simulink subsystem "ConfiguredSimulinkPlantModel"  (R2025b)
settings: Solver=VariableStepAuto  StartTime=0.0  StopTime=10.0  RelTol=1e-3
undefined symbols (not defined in the file or in its folder): PlntTrnsfrCaseAxlSpdLock, PlntTrnsfrCaseTrqSplitRatio
libraries: simulink x2
settings Model: ModifiedByFormat=The MathWorks, Inc.  Creator=The MathWorks, Inc.  LastModifiedBy=The MathWorks, Inc.
settings RTWCC: GPUComputeCapability=3.5

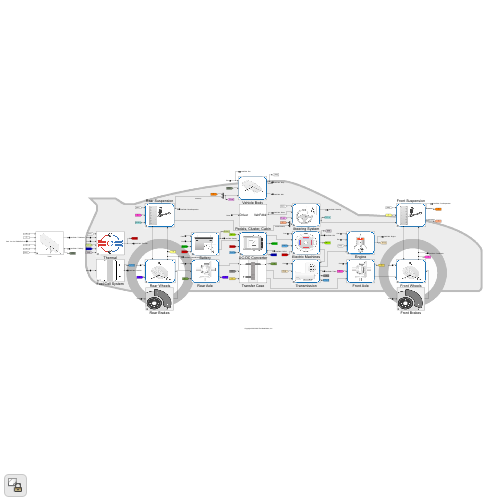
[thumbnail: Simulink's stored preview of the top-level diagram]
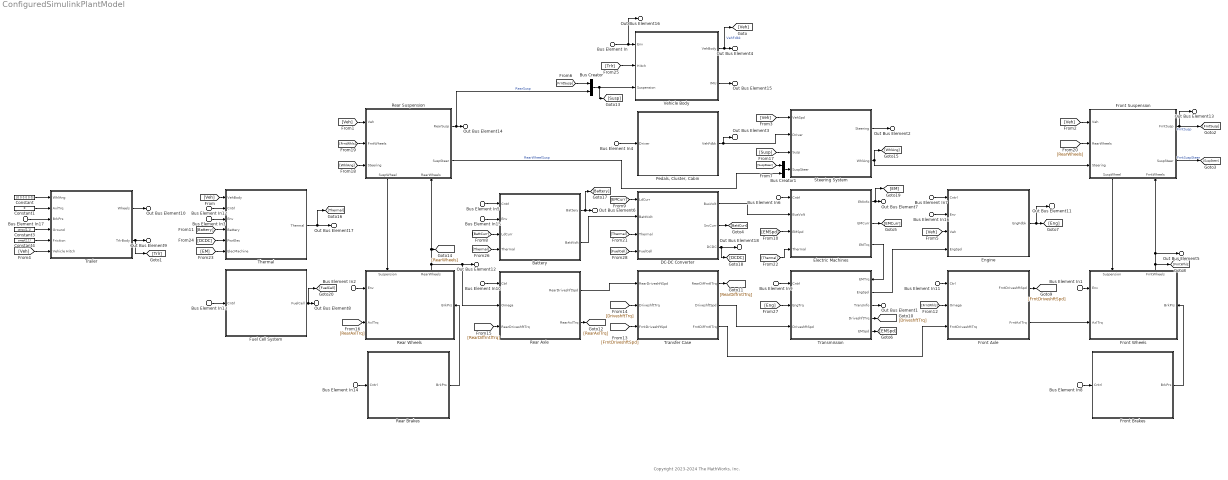
== system ConfiguredSimulinkPlantModel ==
  note: Copyright 2023-2024 The MathWorks, Inc.
  Bus Element In{,1..3,15..16} (6 alike) : Inport  PortName=Env
  Bus Element In4 : Inport  Port=2  PortName=Driver
  Bus Element In{5..14} (10 alike) : Inport  Port=3  PortName=Cntrl
  Bus Element In17 : Inport  Port=3  PortName=Cntrl  Element=Vcu.VcuTrlrBrkPrsCmd
  Battery : Subsystem  Variant=on  VariantChoicesSpecifier={'BatteryMapped'}  VariantControlMode=label  VariantControl=Battery  LabelModeActiveChoice=BatteryMapped
      mask Display: image('Battery.png'); % Use "Edit Image" on toolstrip to change.
  Bus Creator : BusCreator  Inputs=2
  Bus Creator1 : BusCreator  Inputs=2
  Constant : Constant  Value=[0 0 0 0 0 0]
  Constant1 : Constant  Value=0
  Constant3 : Constant  Value=zeros(2,1)
  Constant4 : Constant  Value=ones(2,1)
  DC-DC Converter : Subsystem  Variant=on  VariantChoicesSpecifier={'HVDCPassThrough'}  VariantControlMode=label  VariantControl=DC-DC Converter  LabelModeActiveChoice=HVDCPassThrough
      mask Display: image('DCDCConverter.png'); % Use "Edit Image" on toolstrip to change.
  Electric Machines : Subsystem  Variant=on  VariantChoicesSpecifier={'s2EM'}  VariantControlMode=label  VariantControl=Electric Machines  LabelModeActiveChoice=s2EM
      mask Display: image('Motor.png'); % Use "Edit Image" on toolstrip to change.
  Engine : Subsystem  Variant=on  VariantChoicesSpecifier={'SiMappedEngine'}  VariantControlMode=label  VariantControl=Engine  LabelModeActiveChoice=SiMappedEngine
      mask Display: image('Engine.png');
  Front Axle : Subsystem
      mask Display: image('OpenDifferential.png');
  Front Brakes : Subsystem  Variant=on  VariantControlMode=label  LabelModeActiveChoice=BrakingHydraulics
      mask Display: image('Caliper.png');
  Front Suspension : Subsystem  Variant=on  VariantChoicesSpecifier={'NoSuspensionFront'}  VariantControlMode=label  VariantControl=Front Suspension  LabelModeActiveChoice=NoSuspensionFront
      settings: PortSchema="{\"entries\":[{\"content\":{\"sides\":[{\"content\":{\"connectorIds\":[\"In1\",\"In2\",\"In3\"]},\"type\":\"ConnectorPlacement.EquallySpacedRectSide\",\"uuid\":\"03d471f7-20fa-4f88-95ae-1ed5ac0b2add\"},{\"content\":{\"connectorIds\":[\"Out1\",\"Out2\"],\"side\":\"RIGHT\"},\"type\":\"ConnectorPlacement.EquallySpacedRectSide\",\"uuid\":\"9ad6c778-1a7a-40eb-a466-797c67a1b13b\"},{\"content\":{\"side\":\"TOP\"},\"type\":\"ConnectorPlacement.EquallySpacedRectSide\",\"uuid\":\"82e0e713-e0a4-4b6c-9efd-1ca5e9a7cc75\"},{\"content\":{\"connectorIds\":[\"Out3\",\"In4\"],\"side\":\"BOTTOM\"},\"type\":\"ConnectorPlacement.EquallySpacedRectSide\",\"uuid\":\"217f9025-16e9-443b-9e91-f4a978a2b175\"}]},\"type\":\"ConnectorPlacement.EquallySpacedConnector\",\"uuid\":\"962b9c26-d5a5-4e4a-bd3b-22a258cb5c30\"}],\"packageUris\":[\"http://schema.mathworks.com/mf0/Connector/R2020b\"],\"version\":\"1.0\"}"
      mask Display: image('SimpleSusp.png'); % Use "Edit Image" on toolstrip to change.
  Front Wheels : Subsystem  Variant=on  VariantChoicesSpecifier={'MFTiresLongitudinalFront'}  VariantControlMode=label  VariantControl=Front Wheels  LabelModeActiveChoice=MFTiresLongitudinalFront
      settings: PortSchema="{\"entries\":[{\"content\":{\"sides\":[{\"content\":{\"connectorIds\":[\"In1\",\"In2\"]},\"type\":\"ConnectorPlacement.EquallySpacedRectSide\",\"uuid\":\"acc304d9-256c-4d8c-a59c-fdc4678acde8\"},{\"content\":{\"connectorIds\":[\"In4\"],\"side\":\"RIGHT\"},\"type\":\"ConnectorPlacement.EquallySpacedRectSide\",\"uuid\":\"17734490-d6e0-42a1-ab4b-fb468dc96262\"},{\"content\":{\"connectorIds\":[\"In3\",\"Out1\"],\"side\":\"TOP\"},\"type\":\"ConnectorPlacement.EquallySpacedRectSide\",\"uuid\":\"b3a5b678-2424-47a9-9e4a-20883a25a01f\"}]},\"type\":\"ConnectorPlacement.EquallySpacedConnector\",\"uuid\":\"2051c4aa-303b-4f53-baee-0d5c16c2d89d\"}],\"packageUris\":[\"http://schema.mathworks.com/mf0/Connector/R2020b\"],\"version\":\"1.0\"}"
      mask Display: image('TirewithNoneBrake.png'); % Use "Edit Image" on toolstrip to change.
  Fuel Cell System : Subsystem  Variant=on  VariantControlMode=label  LabelModeActiveChoice=NoFuelCell
      mask Display: image('FuelCell.png');
  "Pedals, Cluster, Cabin" : Subsystem
  Rear Axle : Subsystem
      mask Display: image('OpenDifferential.png');
  Rear Brakes : Subsystem  Variant=on  VariantControlMode=label  LabelModeActiveChoice=BrakingHydraulics
      mask Display: image('Caliper.png');
  Rear Suspension : Subsystem  Variant=on  VariantChoicesSpecifier={'NoSuspensionRear'}  VariantControlMode=label  VariantControl=Rear Suspension  LabelModeActiveChoice=NoSuspensionRear
      settings: PortSchema="{\"entries\":[{\"content\":{\"sides\":[{\"content\":{\"connectorIds\":[\"In1\",\"In2\",\"In3\"]},\"type\":\"ConnectorPlacement.EquallySpacedRectSide\",\"uuid\":\"7e1e6507-37b6-4974-9884-9358adf4f829\"},{\"content\":{\"connectorIds\":[\"Out1\",\"Out2\"],\"side\":\"RIGHT\"},\"type\":\"ConnectorPlacement.EquallySpacedRectSide\",\"uuid\":\"94f7267b-d499-4c4a-96d7-426dfd795072\"},{\"content\":{\"side\":\"TOP\"},\"type\":\"ConnectorPlacement.EquallySpacedRectSide\",\"uuid\":\"1840464c-d7a2-4658-8971-9ed60c7fc03f\"},{\"content\":{\"connectorIds\":[\"Out3\",\"In4\"],\"side\":\"BOTTOM\"},\"type\":\"ConnectorPlacement.EquallySpacedRectSide\",\"uuid\":\"eeb43409-2567-47b0-b34c-ce9f28d6ee5f\"}]},\"type\":\"ConnectorPlacement.EquallySpacedConnector\",\"uuid\":\"348a381a-4a9d-4c35-9a3c-c7ca8ef0f246\"}],\"packageUris\":[\"http://schema.mathworks.com/mf0/Connector/R2020b\"],\"version\":\"1.0\"}"
      mask Display: image('SimpleSusp.png'); % Use "Edit Image" on toolstrip to change.
  Rear Wheels : Subsystem  Variant=on  VariantChoicesSpecifier={'MFTiresLongitudinalRear'}  VariantControlMode=label  VariantControl=Rear Wheels  LabelModeActiveChoice=MFTiresLongitudinalRear
      settings: PortSchema="{\"entries\":[{\"content\":{\"sides\":[{\"content\":{\"connectorIds\":[\"In1\",\"In2\"]},\"type\":\"ConnectorPlacement.EquallySpacedRectSide\",\"uuid\":\"acc304d9-256c-4d8c-a59c-fdc4678acde8\"},{\"content\":{\"connectorIds\":[\"In4\"],\"side\":\"RIGHT\"},\"type\":\"ConnectorPlacement.EquallySpacedRectSide\",\"uuid\":\"17734490-d6e0-42a1-ab4b-fb468dc96262\"},{\"content\":{\"connectorIds\":[\"In3\",\"Out1\"],\"side\":\"TOP\"},\"type\":\"ConnectorPlacement.EquallySpacedRectSide\",\"uuid\":\"b3a5b678-2424-47a9-9e4a-20883a25a01f\"}]},\"type\":\"ConnectorPlacement.EquallySpacedConnector\",\"uuid\":\"2051c4aa-303b-4f53-baee-0d5c16c2d89d\"}],\"packageUris\":[\"http://schema.mathworks.com/mf0/Connector/R2020b\"],\"version\":\"1.0\"}"
      mask Display: image('TirewithNoneBrake.png'); % Use "Edit Image" on toolstrip to change.
  Steering System : Subsystem  Variant=on  VariantChoicesSpecifier={'NoSteering'}  VariantControlMode=label  VariantControl=Steering System  LabelModeActiveChoice=NoSteering
      mask Display: image('SteeringSystemicon.png'); % Use "Edit Image" on toolstrip to change.
  Thermal : Subsystem  Variant=on  VariantChoicesSpecifier={'NoThermalEffect'}  VariantControlMode=label  VariantControl=Thermal  LabelModeActiveChoice=NoThermalEffect
      mask Display: image('ThermalNoFrm.png'); % Use "Edit Image" on toolstrip to change.
  Trailer : Subsystem  Variant=on  VariantChoicesSpecifier={'NoTrailer'}  VariantControlMode=label  VariantControl=No Trailer  LabelModeActiveChoice=NoTrailer
      mask Display: image('6dof1axletrailer.png');
  Transfer Case : Subsystem
      mask Display: image('transfercase.png'); % Use "Edit Image" on toolstrip to change.
  Transmission : Subsystem  Variant=on  VariantChoicesSpecifier={'HEVMM'}  VariantControlMode=label  VariantControl=Transmission  LabelModeActiveChoice=HEVMM
      settings: PortSchema="{\"entries\":[{\"content\":{\"sides\":[{\"content\":{\"connectorIds\":[\"In1\",\"In2\",\"In3\"]},\"type\":\"ConnectorPlacement.EquallySpacedRectSide\",\"uuid\":\"1993136c-9a3a-44ff-911b-f5c4b5f170d3\"},{\"content\":{\"connectorIds\":[\"In4\",\"Out1\",\"Out2\",\"Out3\",\"Out4\"],\"side\":\"RIGHT\"},\"type\":\"ConnectorPlacement.EquallySpacedRectSide\",\"uuid\":\"aff4cb27-7ab4-4732-ab7d-c92ab59c9626\"},{\"content\":{\"side\":\"TOP\"},\"type\":\"ConnectorPlacement.EquallySpacedRectSide\",\"uuid\":\"ab1ce95b-6219-4ec3-a6c3-82db85a81250\"}]},\"type\":\"ConnectorPlacement.EquallySpacedConnector\",\"uuid\":\"efacb2a6-e0ab-499c-b572-ed8cdbf6ceba\"}],\"packageUris\":[\"http://schema.mathworks.com/mf0/Connector/R2020b\"],\"version\":\"1.0\"}"
      mask Display: image('Transmission.png'); % Use "Edit Image" on toolstrip to change.
  Vehicle Body : Subsystem
      mask Display: image('VehDynLat.png');
  Out Bus Element3 : Outport  PortName=VehFdbk  Element=Driver
  Out Bus Element4 : Outport  PortName=VehFdbk  Element=Body
  Out Bus Element5 : Outport  PortName=VehFdbk  Element=FrntWheels
  Out Bus Element1 : Outport  PortName=VehFdbk  Element=Trans
  Out Bus Element2 : Outport  PortName=VehFdbk  Element=Steering
  Out Bus Element6 : Outport  PortName=VehFdbk  Element=Battery
  Out Bus Element7 : Outport  PortName=VehFdbk  Element=EM
  Out Bus Element8 : Outport  PortName=VehFdbk  Element=FuelCell
  Out Bus Element11 : Outport  PortName=VehFdbk  Element=Engine
  Out Bus Element13 : Outport  PortName=VehFdbk  Element=FrntSuspension
  Out Bus Element9 : Outport  PortName=VehFdbk  Element=TrlrBody
  Out Bus Element10 : Outport  PortName=VehFdbk  Element=TrlrWheels
  Out Bus Element12 : Outport  PortName=VehFdbk  Element=RearWheels
  Out Bus Element14 : Outport  PortName=VehFdbk  Element=RearSuspension
  Out Bus Element15 : Outport  PortName=VehFdbk  Element=IMU
  Out Bus Element16 : Outport  PortName=VehFdbk  Element=Env
  Out Bus Element17 : Outport  PortName=VehFdbk  Element=Thermal
  Out Bus Element18 : Outport  PortName=VehFdbk  Element=DCDC
  wires:
  Bus Element In4/1 -> "Pedals, Cluster, Cabin"/1(Driver)
  Bus Element In12/1 -> Thermal/2(Cntrl)
  Bus Element In14/1 -> Rear Brakes/1(Cntrl)
  Electric Machines/1(EMInfo) -> Out Bus Element7/1, [EM]
  Front Brakes/1(BrkPrs) -> Front Wheels/4(BrkPrs)
  Rear Brakes/1(BrkPrs) -> Rear Wheels/4(BrkPrs)
  Rear Wheels/1(RearWheels) -> Rear Axle/2(Omega), Out Bus Element12/1, Rear Suspension/4(RearWheels), [RearWheels]
  Engine/1(EngFdbk) -> Out Bus Element11/1, [Eng]
  Bus Element In7/1 -> Engine/1(Cntrl)
  Front Suspension/1(FrntSusp) -> Out Bus Element13/1, [FrntSusp]  "FrntSusp"
  Bus Element In8/1 -> Front Brakes/1(Cntrl)
  "Pedals, Cluster, Cabin"/1(VehFdbk) -> Out Bus Element3/1, Steering System/2(Driver)
  Vehicle Body/2(IMU) -> Out Bus Element15/1
  Bus Element In2/1 -> Rear Wheels/1(Env)
  Bus Element In3/1 -> Thermal/3(Env)
  Front Wheels/1(FrntWheels) -> [FrntWhls], Out Bus Element5/1, Front Suspension/4(FrntWheels)
  Bus Element In13/1 -> Fuel Cell System/1(Cntrl)
  [Trlr] -> Vehicle Body/2(Hitch)
  Bus Element In/1 -> Vehicle Body/1(Env), Out Bus Element16/1
  [Veh] -> Steering System/1(VehSpd)
  Bus Element In11/1 -> Front Axle/1(Ctrl)
  [Veh] -> Front Suspension/1(Veh)
  Trailer/2(TrlrBody) -> Out Bus Element9/1, [Trlr]
  [Veh] -> Rear Suspension/1(Veh)
  [Veh] -> Thermal/1(VehBody)
  Vehicle Body/1(VehBody) -> Out Bus Element4/1, [Veh]  "VehFdbk"
  Trailer/1(Wheels) -> Out Bus Element10/1
  Rear Suspension/1(RearSusp) -> Out Bus Element14/1, Bus Creator/2  "RearSusp"
  Transmission/2(TransInfo) -> Out Bus Element1/1
  Fuel Cell System/1(FuelCell) -> [FuelCell], Out Bus Element8/1
  Thermal/1(Thermal) -> Out Bus Element17/1, [Thermal]
  Bus Element In9/1 -> Transmission/1(Cntrl)
  Bus Element In1/1 -> Front Wheels/1(Env)
  Bus Element In5/1 -> Battery/1(Cntrl)
  Battery/1(Battery) -> Out Bus Element6/1, [Battery]
  Bus Element In6/1 -> Electric Machines/1(Cntrl)
  Steering System/1(Steering) -> Out Bus Element2/1
  [FrntSusp] -> Bus Creator/1
  Front Suspension/3(SuspWheel) -> Front Wheels/3(Suspension)
  Rear Suspension/3(SuspWheel) -> Rear Wheels/3(Suspension)
  Rear Suspension/2(SuspSteer) -> Bus Creator1/2  "RearWheelSusp"
  Front Suspension/2(SuspSteer) -> [SuspSteer]  "FrntSuspSteer"
  Battery/2(BattVolt) -> DC-DC Converter/2(BattVolt)
  DC-DC Converter/1(BusVolt) -> Electric Machines/2(BusVolt)
  DC-DC Converter/2(SrcCurr) -> [BattCurr]
  Bus Element In10/1 -> Rear Axle/1(Ctrl)
  Transfer Case/2(DriveshftSpd) -> Transmission/3(DriveshftSpd)
  Electric Machines/3(EMTrq) -> Transmission/4(EMTrq)
  Transmission/3(DriveshftTrq) -> [DriveshftTrq]
  Transfer Case/3(FrntDiffrntlTrq) -> Front Axle/3(FrntDriveshftTrq)
  Transfer Case/1(RearDiffrntlTrq) -> [RearDiffrntlTrq]
  Front Axle/1(FrntDriveshftSpd) -> [FrntDriveshftSpd]
  Rear Axle/1(RearDriveshftSpd) -> Transfer Case/1(RearDriveshftSpd)
  Front Axle/2(FrntAxlTrq) -> Front Wheels/2(AxlTrq)
  Rear Axle/2(RearAxlTrq) -> [RearAxlTrq]
  Transmission/4(EMSpd) -> [EMSpd]
  Bus Element In15/1 -> Battery/2(Env)
  Transmission/1(EngSpd) -> Engine/4(EngSpd)
  Bus Element In16/1 -> Engine/2(Env)
  [Veh] -> Engine/3(Veh)
  [SuspSteer] -> Bus Creator1/1
  [BattCurr] -> Battery/3(LdCurr)
  Electric Machines/2(EMCurr) -> [EMCurr]
  [EMCurr] -> DC-DC Converter/1(LdCurr)
  [EMSpd] -> Electric Machines/3(EMSpd)
  [Eng] -> Transmission/2(EngTrq)
  [FrntWhls] -> Front Axle/2(Omega)
  [FrntDriveshftSpd] -> Transfer Case/3(FrntDriveshftSpd)
  [DriveshftTrq] -> Transfer Case/2(DriveshftTrq)
  [RearDiffrntlTrq] -> Rear Axle/3(RearDriveshftTrq)
  [RearAxlTrq] -> Rear Wheels/2(AxlTrq)
  Bus Creator1/1 -> Steering System/4(SuspSteer)
  [Susp] -> Steering System/3(Susp)
  [RearWheels] -> Front Suspension/2(RearWheels)
  [FrntWhls] -> Rear Suspension/2(FrntWheels)
  Steering System/2(WhlAng) -> [WhlAng], Front Suspension/3(Steering)
  Bus Creator/1 -> Vehicle Body/3(Suspension), [Susp]
  [WhlAng] -> Rear Suspension/3(Steering)
  DC-DC Converter/3(DCDC) -> Out Bus Element18/1, [DCDC]
  [Thermal] -> DC-DC Converter/3(Thermal)
  [Thermal] -> Electric Machines/4(Thermal)
  [Battery] -> Thermal/4(Battery)
  [DCDC] -> Thermal/5(PwrElec)
  [EM] -> Thermal/6(ElecMachine)
  [Thermal] -> Battery/4(Thermal)
  Constant4/1 -> Trailer/5(Friction)
  Constant/1 -> Trailer/1(WhlAng)
  Constant3/1 -> Trailer/4(Ground)
  [Veh] -> Trailer/6(Vehicle Hitch)
  Bus Element In17/1 -> Trailer/3(BrkPrs)
  Constant1/1 -> Trailer/2(AxlTrq)
  [FuelCell] -> DC-DC Converter/4(FuelCell)

== system ConfiguredSimulinkPlantModel/Battery ==
  Cntrl : Inport
  Env : Inport  Port=2
  LdCurr : Inport  Port=3
  Thermal : Inport  Port=4
  BatteryMapped : Subsystem  VariantControl=BatteryMapped  ReferencedSubsystem=BatteryMapped
  Battery : Outport
  BattVolt : Outport  Port=2

== system ConfiguredSimulinkPlantModel/DC-DC Converter ==
  LdCurr : Inport
  BattVolt : Inport  Port=2
  Thermal : Inport  Port=3
  FuelCell : Inport  Port=4
  HVDCPassThrough : Subsystem  VariantControl=HVDCPassThrough  ReferencedSubsystem=HVDCPassThrough
  BusVolt : Outport
  SrcCurr : Outport  Port=2
  DCDC : Outport  Port=3

== system ConfiguredSimulinkPlantModel/Electric Machines ==
  Cntrl : Inport
  BusVolt : Inport  Port=2
  EMSpd : Inport  Port=3
  Thermal : Inport  Port=4
  s2EM : Subsystem  VariantControl=s2EM  ReferencedSubsystem=s2EM
  EMInfo : Outport
  EMCurr : Outport  Port=2
  EMTrq : Outport  Port=3

== system ConfiguredSimulinkPlantModel/Engine ==
  Cntrl : Inport
  Env : Inport  Port=2
  Veh : Inport  Port=3
  EngSpd : Inport  Port=4
  SiMappedEngine : Subsystem  VariantControl=SiMappedEngine  ReferencedSubsystem=SiMappedEngine
  EngFdbk : Outport

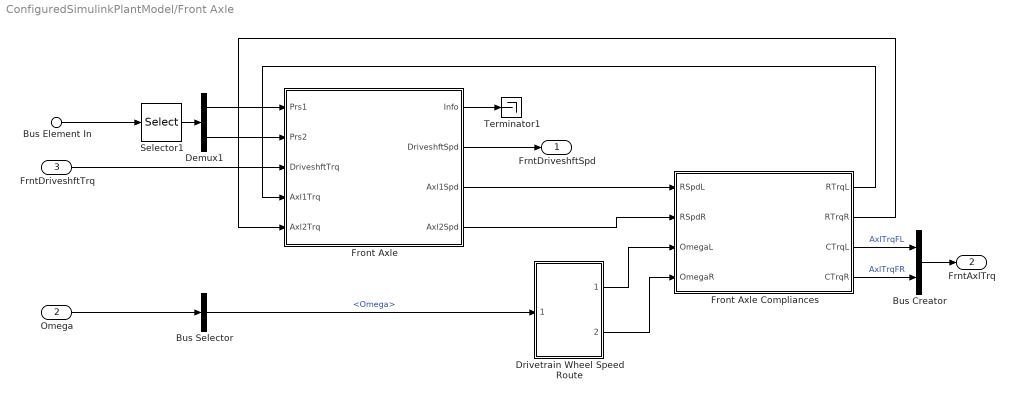
== system ConfiguredSimulinkPlantModel/Front Axle ==
  Bus Element In : Inport  PortName=Ctrl  Element=Diff.DiffrntlPrsCmd
  Omega : Inport  Port=2
  FrntDriveshftTrq : Inport  Port=3
  Bus Creator : BusCreator  Inputs=2
  Bus Selector : BusSelector  OutputSignals=Wheels.Omega
  Demux1 : Demux  Outputs=2
  Drivetrain Wheel Speed Route : Subsystem  Variant=on  VariantControlMode=label  LabelModeActiveChoice=Bus
  Front Axle : Subsystem  Variant=on  VariantChoicesSpecifier={'OpenDifferential'}  VariantControlMode=label  VariantControl=Choice  LabelModeActiveChoice=OpenDifferential
  Front Axle Compliances : Subsystem  Variant=on  VariantChoicesSpecifier={'AxleCompliances'}  VariantControlMode=label  VariantControl=Choice  LabelModeActiveChoice=AxleCompliances
  Selector1 : Selector  InputPortWidth=4  IndexOptions=Index vector (dialog)  Indices=[1 2]  OutputSizes=1
  Terminator1 : Terminator
  FrntDriveshftSpd : Outport
  FrntAxlTrq : Outport  Port=2
  wires:
  Bus Creator/1 -> FrntAxlTrq/1
  Omega/1 -> Bus Selector/1
  Drivetrain Wheel Speed Route/2(Omega_FR) -> Front Axle Compliances/4(OmegaR)
  Demux1/1 -> Front Axle/1(Prs1)
  Selector1/1 -> Demux1/1
  Front Axle Compliances/1(RTrqL) -> Front Axle/4(Axl1Trq)
  Bus Selector/1 -> Drivetrain Wheel Speed Route/1(Omega)  "<Omega>"
  Bus Element In/1 -> Selector1/1
  Front Axle Compliances/2(RTrqR) -> Front Axle/5(Axl2Trq)
  Front Axle/3(Axl1Spd) -> Front Axle Compliances/1(RSpdL)
  Front Axle/4(Axl2Spd) -> Front Axle Compliances/2(RSpdR)
  Demux1/2 -> Front Axle/2(Prs2)
  Front Axle Compliances/3(CTrqL) -> Bus Creator/1  "AxlTrqFL"
  Front Axle/1(Info) -> Terminator1/1
  FrntDriveshftTrq/1 -> Front Axle/3(DriveshftTrq)
  Front Axle/2(DriveshftSpd) -> FrntDriveshftSpd/1
  Front Axle Compliances/4(CTrqR) -> Bus Creator/2  "AxlTrqFR"
  Drivetrain Wheel Speed Route/1(Omega_FL) -> Front Axle Compliances/3(OmegaL)

== system ConfiguredSimulinkPlantModel/Front Brakes ==
  Cntrl : Inport
  BrakingHydraulics : Subsystem  VariantControl=BrakingHydraulics  ReferencedSubsystem=BrakingHydraulics
  BrkPrs : Outport

== system ConfiguredSimulinkPlantModel/Front Suspension ==
  Veh : Inport
  RearWheels : Inport  Port=2
  Steering : Inport  Port=3
  FrntWheels : Inport  Port=4
  NoSuspensionFront : Subsystem  VariantControl=NoSuspensionFront  ReferencedSubsystem=NoSuspensionFront
  FrntSusp : Outport
  SuspSteer : Outport  Port=2
  SuspWheel : Outport  Port=3

== system ConfiguredSimulinkPlantModel/Front Wheels ==
  Env : Inport
  AxlTrq : Inport  Port=2
  Suspension : Inport  Port=3
  BrkPrs : Inport  Port=4
  MFTiresLongitudinalFront : Subsystem  VariantControl=MFTiresLongitudinalFront  ReferencedSubsystem=MFTiresLongitudinalFront
  FrntWheels : Outport

== system ConfiguredSimulinkPlantModel/Fuel Cell System ==
  Cntrl : Inport
  NoFuelCell : Subsystem  VariantControl=NoFuelCell  ReferencedSubsystem=NoFuelCell
  FuelCell : Outport

== system ConfiguredSimulinkPlantModel/Pedals, Cluster, Cabin ==
  Driver : Inport
  Pedal Cluster Input : Subsystem
  "Pedal, Cluster, Cabin" : Subsystem
  VehFdbk : Outport
  wires:
  "Pedal, Cluster, Cabin"/1(Driver) -> VehFdbk/1
  Driver/1 -> Pedal Cluster Input/1(Driver)
  Pedal Cluster Input/10(HazzardCmd) -> "Pedal, Cluster, Cabin"/10(HazzardCmd)
  Pedal Cluster Input/9(RightSignalCmd) -> "Pedal, Cluster, Cabin"/9(RightSignalCmd)
  Pedal Cluster Input/8(LeftSignalCmd) -> "Pedal, Cluster, Cabin"/8(LeftSignalCmd)
  Pedal Cluster Input/7(LowBeamCmd) -> "Pedal, Cluster, Cabin"/7(LowBeamCmd)
  Pedal Cluster Input/6(HighBeamCmd) -> "Pedal, Cluster, Cabin"/6(HighBeamCmd)
  Pedal Cluster Input/5(IgnCmd) -> "Pedal, Cluster, Cabin"/5(IgCmd)
  Pedal Cluster Input/4(DrvrGearCmd) -> "Pedal, Cluster, Cabin"/4(GearCmd)
  Pedal Cluster Input/3(DecelCmd) -> "Pedal, Cluster, Cabin"/3(DecelCmd)
  Pedal Cluster Input/2(AccelCmd) -> "Pedal, Cluster, Cabin"/2(AccCmd)
  Pedal Cluster Input/1(SteerCmd) -> "Pedal, Cluster, Cabin"/1(SteerCmd)

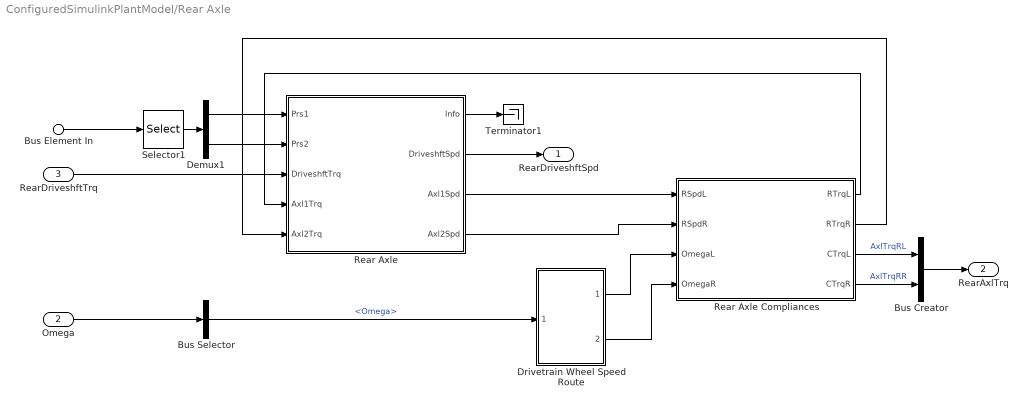
== system ConfiguredSimulinkPlantModel/Rear Axle ==
  Bus Element In : Inport  PortName=Ctrl  Element=Diff.DiffrntlPrsCmd
  Omega : Inport  Port=2
  RearDriveshftTrq : Inport  Port=3
  Bus Creator : BusCreator  Inputs=2
  Bus Selector : BusSelector  OutputSignals=Wheels.Omega
  Demux1 : Demux  Outputs=2
  Drivetrain Wheel Speed Route : Subsystem  Variant=on  VariantControlMode=label  LabelModeActiveChoice=Bus
  Rear Axle : Subsystem  Variant=on  VariantChoicesSpecifier={'NoDifferential'}  VariantControlMode=label  VariantControl=Choice  LabelModeActiveChoice=NoDifferential
  Rear Axle Compliances : Subsystem  Variant=on  VariantChoicesSpecifier={'NoAxleCompliances'}  VariantControlMode=label  VariantControl=Choice  LabelModeActiveChoice=NoAxleCompliances
  Selector1 : Selector  InputPortWidth=4  IndexOptions=Index vector (dialog)  Indices=[3 4]  OutputSizes=1
  Terminator1 : Terminator
  RearDriveshftSpd : Outport
  RearAxlTrq : Outport  Port=2
  wires:
  Omega/1 -> Bus Selector/1
  Rear Axle/3(Axl1Spd) -> Rear Axle Compliances/1(RSpdL)
  Rear Axle Compliances/4(CTrqR) -> Bus Creator/2  "AxlTrqRR"
  Rear Axle/1(Info) -> Terminator1/1
  Rear Axle Compliances/2(RTrqR) -> Rear Axle/5(Axl2Trq)
  Rear Axle Compliances/1(RTrqL) -> Rear Axle/4(Axl1Trq)
  Rear Axle Compliances/3(CTrqL) -> Bus Creator/1  "AxlTrqRL"
  Rear Axle/2(DriveshftSpd) -> RearDriveshftSpd/1
  Drivetrain Wheel Speed Route/1(Omega_RL) -> Rear Axle Compliances/3(OmegaL)
  Rear Axle/4(Axl2Spd) -> Rear Axle Compliances/2(RSpdR)
  Selector1/1 -> Demux1/1
  Drivetrain Wheel Speed Route/2(Omega_RR) -> Rear Axle Compliances/4(OmegaR)
  RearDriveshftTrq/1 -> Rear Axle/3(DriveshftTrq)
  Demux1/1 -> Rear Axle/1(Prs1)
  Demux1/2 -> Rear Axle/2(Prs2)
  Bus Selector/1 -> Drivetrain Wheel Speed Route/1(Omega)  "<Omega>"
  Bus Creator/1 -> RearAxlTrq/1
  Bus Element In/1 -> Selector1/1

== system ConfiguredSimulinkPlantModel/Rear Brakes ==
  Cntrl : Inport
  BrakingHydraulics : Subsystem  VariantControl=BrakingHydraulics  ReferencedSubsystem=BrakingHydraulics
  BrkPrs : Outport

== system ConfiguredSimulinkPlantModel/Rear Suspension ==
  Veh : Inport
  FrntWheels : Inport  Port=2
  Steering : Inport  Port=3
  RearWheels : Inport  Port=4
  NoSuspensionRear : Subsystem  VariantControl=NoSuspensionRear  ReferencedSubsystem=NoSuspensionRear
  RearSusp : Outport
  SuspSteer : Outport  Port=2
  SuspWheel : Outport  Port=3

== system ConfiguredSimulinkPlantModel/Rear Wheels ==
  Env : Inport
  AxlTrq : Inport  Port=2
  Suspension : Inport  Port=3
  BrkPrs : Inport  Port=4
  MFTiresLongitudinalRear : Subsystem  VariantControl=MFTiresLongitudinalRear  ReferencedSubsystem=MFTiresLongitudinalRear
  RearWheels : Outport

== system ConfiguredSimulinkPlantModel/Steering System ==
  VehSpd : Inport
  Driver : Inport  Port=2
  Susp : Inport  Port=3
  SuspSteer : Inport  Port=4
  NoSteering : Subsystem  VariantControl=NoSteering  ReferencedSubsystem=NoSteering
  Steering : Outport
  WhlAng : Outport  Port=2

== system ConfiguredSimulinkPlantModel/Thermal ==
  VehBody : Inport
  Cntrl : Inport  Port=2
  Env : Inport  Port=3
  Battery : Inport  Port=4
  PwrElec : Inport  Port=5
  ElecMachine : Inport  Port=6
  NoThermalEffect : Subsystem  VariantControl=NoThermalEffect  ReferencedSubsystem=NoThermalEffect
  Thermal : Outport

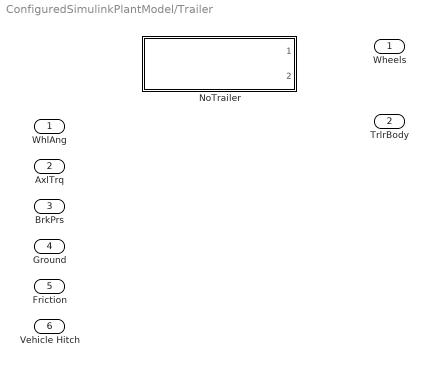
== system ConfiguredSimulinkPlantModel/Trailer ==
  WhlAng : Inport
  AxlTrq : Inport  Port=2
  BrkPrs : Inport  Port=3
  Ground : Inport  Port=4
  Friction : Inport  Port=5
  Vehicle Hitch : Inport  Port=6
  NoTrailer : Subsystem  VariantControl=NoTrailer  ReferencedSubsystem=NoTrailer
  Wheels : Outport
  TrlrBody : Outport  Port=2

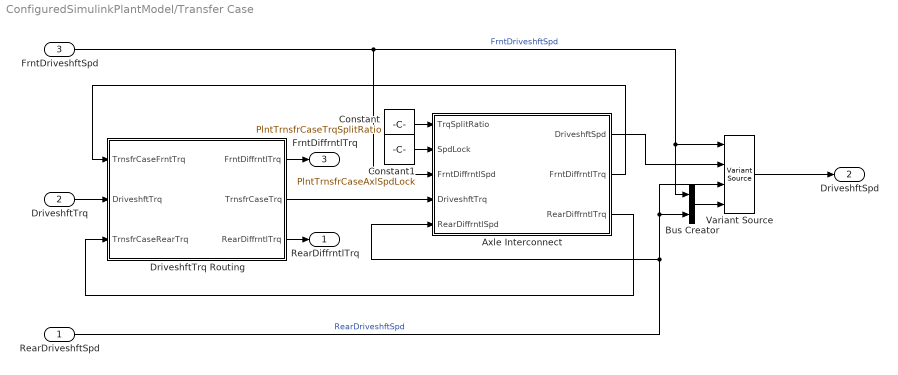
== system ConfiguredSimulinkPlantModel/Transfer Case ==
  RearDriveshftSpd : Inport
  DriveshftTrq : Inport  Port=2
  FrntDriveshftSpd : Inport  Port=3
  Axle Interconnect : Subsystem  Variant=on  VariantChoicesSpecifier={'NoInterconnect'}  VariantControlMode=label  VariantControl=Choice  LabelModeActiveChoice=NoInterconnect
  Bus Creator : BusCreator  Inputs=2
  Constant : Constant  Value=PlntTrnsfrCaseTrqSplitRatio  SampleTime=-1
  Constant1 : Constant  Value=PlntTrnsfrCaseAxlSpdLock  SampleTime=-1
  DriveshftTrq Routing : Subsystem  Variant=on  VariantChoicesSpecifier={'OneActuatorFWD'}  VariantControlMode=label  VariantControl=Choice  LabelModeActiveChoice=OneActuatorFWD
  Variant Source : VariantSource  VariantControlMode=label  LabelModeActiveChoice=One Actuator FWD  VariantControls={One Actuator FWD, One Actuator AWD, One Actuator RWD, Multi Actuator AWD}
  RearDiffrntlTrq : Outport  VectorParamsAs1DForOutWhenUnconnected=off
  DriveshftSpd : Outport  Port=2  VectorParamsAs1DForOutWhenUnconnected=off
  FrntDiffrntlTrq : Outport  Port=3  VectorParamsAs1DForOutWhenUnconnected=off
  wires:
  DriveshftTrq Routing/3(RearDiffrntlTrq) -> RearDiffrntlTrq/1
  DriveshftTrq Routing/1(FrntDiffrntlTrq) -> FrntDiffrntlTrq/1
  Variant Source/1 -> DriveshftSpd/1
  Axle Interconnect/3(RearDiffrntlTrq) -> DriveshftTrq Routing/3("TrnsfrCaseRearTrq ")
  Axle Interconnect/2(FrntDiffrntlTrq) -> DriveshftTrq Routing/1(TrnsfrCaseFrntTrq)
  RearDriveshftSpd/1 -> Bus Creator/2, Variant Source/3, Axle Interconnect/5(RearDiffrntlSpd)  "RearDriveshftSpd"
  Axle Interconnect/1(DriveshftSpd) -> Variant Source/2
  FrntDriveshftSpd/1 -> Axle Interconnect/3(FrntDiffrntlSpd), Bus Creator/1, Variant Source/1  "FrntDriveshftSpd"
  Bus Creator/1 -> Variant Source/4
  DriveshftTrq Routing/2(TrnsfrCaseTrq) -> Axle Interconnect/4(DriveshftTrq)
  DriveshftTrq/1 -> DriveshftTrq Routing/2(DriveshftTrq)
  Constant/1 -> Axle Interconnect/1(TrqSplitRatio)
  Constant1/1 -> Axle Interconnect/2(SpdLock)

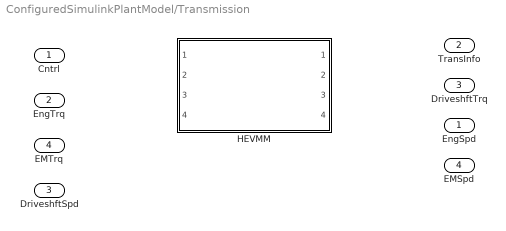
== system ConfiguredSimulinkPlantModel/Transmission ==
  Cntrl : Inport
  EngTrq : Inport  Port=2
  DriveshftSpd : Inport  Port=3
  EMTrq : Inport  Port=4
  HEVMM : Subsystem  VariantControl=HEVMM  ReferencedSubsystem=HEVMM
  EngSpd : Outport
  TransInfo : Outport  Port=2
  DriveshftTrq : Outport  Port=3
  EMSpd : Outport  Port=4

== system ConfiguredSimulinkPlantModel/Vehicle Body ==
  note: Copyright 2022 The MathWorks, Inc.
  Bus Element In : Inport  PortName=Env
  Hitch : Inport  Port=2
  Suspension : Inport  Port=3
  IMu Sensor : Subsystem  Variant=on  VariantChoicesSpecifier={'NoIMUSensor'}  VariantControlMode=label  VariantControl=Choice  LabelModeActiveChoice=NoIMUSensor
  Vehicle : Subsystem  Variant=on  VariantChoicesSpecifier={'VehicleBody3DOFLongitudinal'}  VariantControlMode=label  VariantControl=Vehicle  LabelModeActiveChoice=VehicleBody3DOFLongitudinal
  Bus Element Out : Outport  PortName=VehBody
  Bus Element Out8 : Outport  Port=2  PortName=IMU
  wires:
  Suspension/1 -> Vehicle/1(Suspension)
  Bus Element In/1 -> Vehicle/3(Env)
  IMu Sensor/1(IMU) -> Bus Element Out8/1  "IMU"
  Vehicle/1(VehBody) -> IMu Sensor/1(Veh), Bus Element Out/1
  Hitch/1 -> Vehicle/2(Hitch)

== system ConfiguredSimulinkPlantModel/Front Axle/Drivetrain Wheel Speed Route ==
  Omega : Inport
  Bus : Subsystem  VariantControl=Bus
  Vector : Subsystem  VariantControl=Vector
  Omega_FL : Outport
  Omega_FR : Outport  Port=2

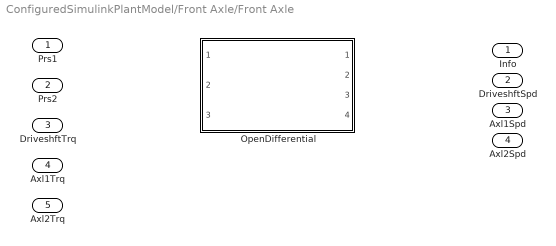
== system ConfiguredSimulinkPlantModel/Front Axle/Front Axle ==
  Prs1 : Inport
  Prs2 : Inport  Port=2
  DriveshftTrq : Inport  Port=3
  Axl1Trq : Inport  Port=4
  Axl2Trq : Inport  Port=5
  OpenDifferential : Subsystem  VariantControl=OpenDifferential  ReferencedSubsystem=OpenDifferential
  Info : Outport
  DriveshftSpd : Outport  Port=2
  Axl1Spd : Outport  Port=3
  Axl2Spd : Outport  Port=4

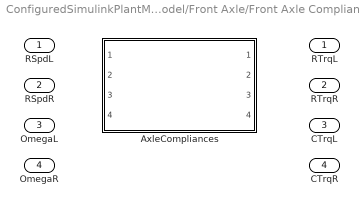
== system ConfiguredSimulinkPlantModel/Front Axle/Front Axle Compliances ==
  RSpdL : Inport
  RSpdR : Inport  Port=2
  OmegaL : Inport  Port=3
  OmegaR : Inport  Port=4
  AxleCompliances : Subsystem  VariantControl=AxleCompliances  ReferencedSubsystem=AxleCompliances
  RTrqL : Outport
  RTrqR : Outport  Port=2
  CTrqL : Outport  Port=3
  CTrqR : Outport  Port=4

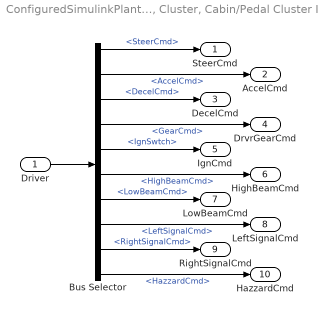
== system ConfiguredSimulinkPlantModel/Pedals, Cluster, Cabin/Pedal Cluster Input ==
  Driver : Inport
  Bus Selector : BusSelector  OutputSignals=SteerCmd,AccelCmd,DecelCmd,GearCmd,IgnSwtch,LightsCmd.HighBeamCmd,LightsCmd.LowBeamCmd,LightsCmd.LeftSignalCmd,LightsCmd.RightSignalCmd,LightsCmd.HazzardCmd
  SteerCmd : Outport  VectorParamsAs1DForOutWhenUnconnected=off
  AccelCmd : Outport  Port=2  VectorParamsAs1DForOutWhenUnconnected=off
  DecelCmd : Outport  Port=3  VectorParamsAs1DForOutWhenUnconnected=off
  DrvrGearCmd : Outport  Port=4  VectorParamsAs1DForOutWhenUnconnected=off
  IgnCmd : Outport  Port=5  VectorParamsAs1DForOutWhenUnconnected=off
  HighBeamCmd : Outport  Port=6  VectorParamsAs1DForOutWhenUnconnected=off
  LowBeamCmd : Outport  Port=7  VectorParamsAs1DForOutWhenUnconnected=off
  LeftSignalCmd : Outport  Port=8  VectorParamsAs1DForOutWhenUnconnected=off
  RightSignalCmd : Outport  Port=9  VectorParamsAs1DForOutWhenUnconnected=off
  HazzardCmd : Outport  Port=10  VectorParamsAs1DForOutWhenUnconnected=off
  wires:
  Bus Selector/2 -> AccelCmd/1  "<AccelCmd>"
  Driver/1 -> Bus Selector/1
  Bus Selector/3 -> DecelCmd/1  "<DecelCmd>"
  Bus Selector/4 -> DrvrGearCmd/1  "<GearCmd>"
  Bus Selector/1 -> SteerCmd/1  "<SteerCmd>"
  Bus Selector/5 -> IgnCmd/1  "<IgnSwtch>"
  Bus Selector/6 -> HighBeamCmd/1  "<HighBeamCmd>"
  Bus Selector/7 -> LowBeamCmd/1  "<LowBeamCmd>"
  Bus Selector/8 -> LeftSignalCmd/1  "<LeftSignalCmd>"
  Bus Selector/9 -> RightSignalCmd/1  "<RightSignalCmd>"
  Bus Selector/10 -> HazzardCmd/1  "<HazzardCmd>"

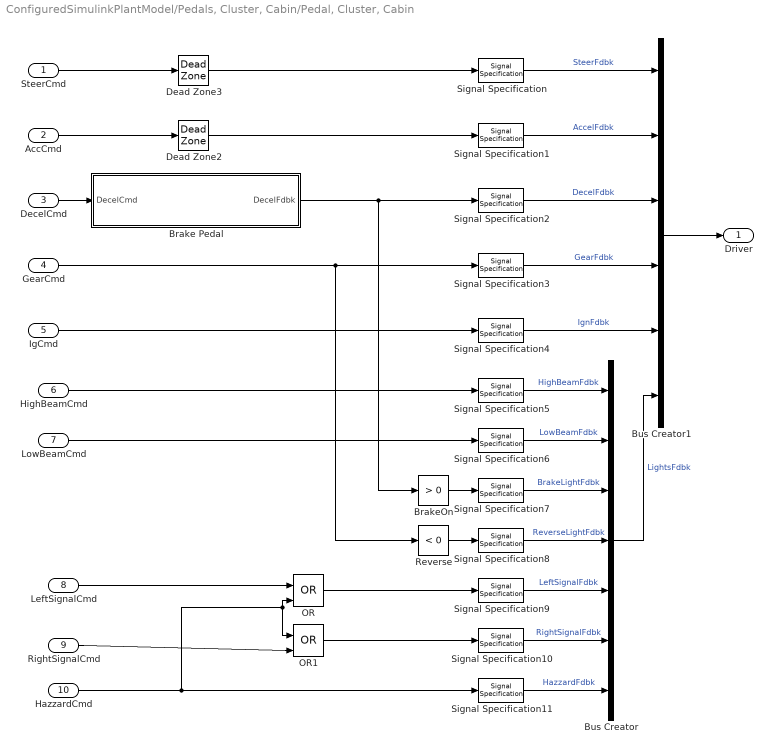
== system ConfiguredSimulinkPlantModel/Pedals, Cluster, Cabin/Pedal, Cluster, Cabin ==
  SteerCmd : Inport
  AccCmd : Inport  Port=2
  DecelCmd : Inport  Port=3
  GearCmd : Inport  Port=4
  IgCmd : Inport  Port=5
  HighBeamCmd : Inport  Port=6
  LowBeamCmd : Inport  Port=7
  LeftSignalCmd : Inport  Port=8
  RightSignalCmd : Inport  Port=9
  HazzardCmd : Inport  Port=10
  Brake Pedal : Subsystem
  BrakeOn : simulink/Logic and Bit Operations/Compare To Constant  relop=>  const=0  OutDataTypeStr=boolean  ZeroCross=off
  Bus Creator : BusCreator  Inputs=7
  Bus Creator1 : BusCreator  Inputs=6
  Dead Zone2 : DeadZone  LowerValue=0  UpperValue=.01  ZeroCross=off
  Dead Zone3 : DeadZone  LowerValue=-.01  UpperValue=.01  ZeroCross=off
  OR : Logic  Operator=OR  IconShape=distinctive  AllPortsSameDT=off  OutDataTypeStr=boolean
  OR1 : Logic  Operator=OR  IconShape=distinctive  AllPortsSameDT=off  OutDataTypeStr=boolean
  Reverse : simulink/Logic and Bit Operations/Compare To Constant  relop=<  const=0  OutDataTypeStr=boolean  ZeroCross=off
  Signal Specification : SignalSpecification  Unit=rad
  Signal Specification{1..11} (11 alike) : SignalSpecification  Unit=1
  Driver : Outport
  wires:
  DecelCmd/1 -> Brake Pedal/1(DecelCmd)
  AccCmd/1 -> Dead Zone2/1
  SteerCmd/1 -> Dead Zone3/1
  Dead Zone2/1 -> Signal Specification1/1
  Signal Specification3/1 -> Bus Creator1/4  "GearFdbk"
  IgCmd/1 -> Signal Specification4/1
  Bus Creator1/1 -> Driver/1
  GearCmd/1 -> Reverse/1, Signal Specification3/1
  Signal Specification2/1 -> Bus Creator1/3  "DecelFdbk"
  Signal Specification/1 -> Bus Creator1/1  "SteerFdbk"
  Brake Pedal/1(DecelFdbk) -> BrakeOn/1, Signal Specification2/1
  Signal Specification4/1 -> Bus Creator1/5  "IgnFdbk"
  Signal Specification1/1 -> Bus Creator1/2  "AccelFdbk"
  Dead Zone3/1 -> Signal Specification/1
  HighBeamCmd/1 -> Signal Specification5/1
  BrakeOn/1 -> Signal Specification7/1
  OR1/1 -> Signal Specification10/1
  OR/1 -> Signal Specification9/1
  Reverse/1 -> Signal Specification8/1
  LeftSignalCmd/1 -> OR/1
  HazzardCmd/1 -> Signal Specification11/1, OR/2, OR1/1
  LowBeamCmd/1 -> Signal Specification6/1
  RightSignalCmd/1 -> OR1/2
  Bus Creator/1 -> Bus Creator1/6  "LightsFdbk"
  Signal Specification5/1 -> Bus Creator/1  "HighBeamFdbk"
  Signal Specification6/1 -> Bus Creator/2  "LowBeamFdbk"
  Signal Specification7/1 -> Bus Creator/3  "BrakeLightFdbk"
  Signal Specification8/1 -> Bus Creator/4  "ReverseLightFdbk"
  Signal Specification10/1 -> Bus Creator/6  "RightSignalFdbk"
  Signal Specification11/1 -> Bus Creator/7  "HazzardFdbk"
  Signal Specification9/1 -> Bus Creator/5  "LeftSignalFdbk"

== system ConfiguredSimulinkPlantModel/Rear Axle/Drivetrain Wheel Speed Route ==
  Omega : Inport
  Bus : Subsystem  VariantControl=Bus
  Vector : Subsystem  VariantControl=Vector
  Omega_RL : Outport
  Omega_RR : Outport  Port=2

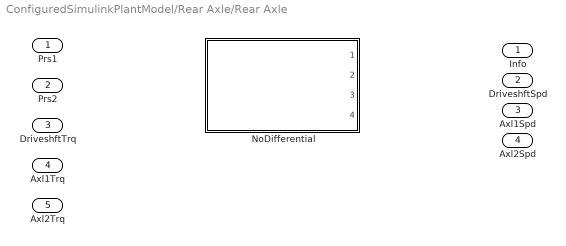
== system ConfiguredSimulinkPlantModel/Rear Axle/Rear Axle ==
  Prs1 : Inport
  Prs2 : Inport  Port=2
  DriveshftTrq : Inport  Port=3
  Axl1Trq : Inport  Port=4
  Axl2Trq : Inport  Port=5
  NoDifferential : Subsystem  VariantControl=NoDifferential  ReferencedSubsystem=NoDifferential
  Info : Outport
  DriveshftSpd : Outport  Port=2
  Axl1Spd : Outport  Port=3
  Axl2Spd : Outport  Port=4

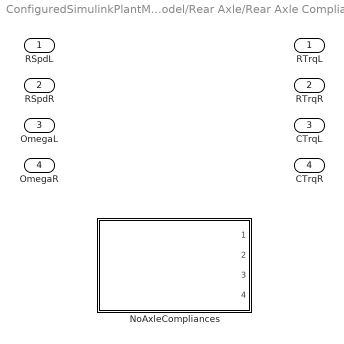
== system ConfiguredSimulinkPlantModel/Rear Axle/Rear Axle Compliances ==
  RSpdL : Inport
  RSpdR : Inport  Port=2
  OmegaL : Inport  Port=3
  OmegaR : Inport  Port=4
  NoAxleCompliances : Subsystem  VariantControl=NoAxleCompliances  ReferencedSubsystem=NoAxleCompliances
  RTrqL : Outport
  RTrqR : Outport  Port=2
  CTrqL : Outport  Port=3
  CTrqR : Outport  Port=4

== system ConfiguredSimulinkPlantModel/Transfer Case/Axle Interconnect ==
  TrqSplitRatio : Inport
  SpdLock : Inport  Port=2
  FrntDiffrntlSpd : Inport  Port=3
  DriveshftTrq : Inport  Port=4
  RearDiffrntlSpd : Inport  Port=5
  NoInterconnect : Subsystem  VariantControl=NoInterconnect  ReferencedSubsystem=NoInterconnect
  DriveshftSpd : Outport
  FrntDiffrntlTrq : Outport  Port=2
  RearDiffrntlTrq : Outport  Port=3

== system ConfiguredSimulinkPlantModel/Transfer Case/DriveshftTrq Routing ==
  TrnsfrCaseFrntTrq : Inport
  DriveshftTrq : Inport  Port=2
  "TrnsfrCaseRearTrq " : Inport  Port=3
  OneActuatorFWD : Subsystem  VariantControl=OneActuatorFWD  ReferencedSubsystem=OneActuatorFWD
  FrntDiffrntlTrq : Outport
  TrnsfrCaseTrq : Outport  Port=2
  RearDiffrntlTrq : Outport  Port=3

== system ConfiguredSimulinkPlantModel/Vehicle Body/IMu Sensor ==
  Veh : Inport
  NoIMUSensor : Subsystem  VariantControl=NoIMUSensor  ReferencedSubsystem=NoIMUSensor
  IMU : Outport

== system ConfiguredSimulinkPlantModel/Vehicle Body/Vehicle ==
  Suspension : Inport
  Hitch : Inport  Port=2
  Env : Inport  Port=3
  VehicleBody3DOFLongitudinal : Subsystem  VariantControl=VehicleBody3DOFLongitudinal  ReferencedSubsystem=VehicleBody3DOFLongitudinal
  VehBody : Outport

== system ConfiguredSimulinkPlantModel/Front Axle/Drivetrain Wheel Speed Route/Bus ==
  Omega : Inport
  Bus Selector1 : BusSelector  OutputSignals=OmegaL,OmegaR
  Omega_FL : Outport
  Omega_FR : Outport  Port=2
  wires:
  Omega/1 -> Bus Selector1/1
  Bus Selector1/1 -> Omega_FL/1  "<OmegaL>"
  Bus Selector1/2 -> Omega_FR/1  "<OmegaR>"

== system ConfiguredSimulinkPlantModel/Front Axle/Drivetrain Wheel Speed Route/Vector ==
  Omega : Inport
  Demux : Demux  Outputs=2
  Omega_FL : Outport
  Omega_FR : Outport  Port=2
  wires:
  Omega/1 -> Demux/1
  Demux/1 -> Omega_FL/1
  Demux/2 -> Omega_FR/1

== system ConfiguredSimulinkPlantModel/Pedals, Cluster, Cabin/Pedal, Cluster, Cabin/Brake Pedal ==
  DecelCmd : Inport
  Dead Zone1 : DeadZone  LowerValue=0  UpperValue=.01  ZeroCross=off
  DecelFdbk : Outport
  wires:
  DecelCmd/1 -> Dead Zone1/1
  Dead Zone1/1 -> DecelFdbk/1

== system ConfiguredSimulinkPlantModel/Rear Axle/Drivetrain Wheel Speed Route/Bus ==
  Omega : Inport
  Bus Selector : BusSelector  OutputSignals=OmegaL,OmegaR
  Omega_RL : Outport
  Omega_RR : Outport  Port=2
  wires:
  Omega/1 -> Bus Selector/1
  Bus Selector/1 -> Omega_RL/1  "<OmegaL>"
  Bus Selector/2 -> Omega_RR/1  "<OmegaR>"

== system ConfiguredSimulinkPlantModel/Rear Axle/Drivetrain Wheel Speed Route/Vector ==
  Omega : Inport
  Demux : Demux  Outputs=2
  Omega_RL : Outport
  Omega_RR : Outport  Port=2
  wires:
  Omega/1 -> Demux/1
  Demux/1 -> Omega_RL/1
  Demux/2 -> Omega_RR/1
